simulink model "ASM_AnimationInterface"  (R2024a)
settings: Solver=ode1  StartTime=SIM.tstart.v  StopTime=SIM.tend.v  FixedStep=SIM.StepSize.v  RelTol=1e-3
PostLoadFcn:
  | , if any(exist('dsrtsu_mdlpostloadfcn', 'file') ~= 0), dsrtsu_mdlpostloadfcn('Execute', bdroot); end,
undefined symbols (not defined in the file): a0b2, b98103fe8ad365046cd0, dsmsi, MDL, SIM
libraries: simulink x22, dsmsilib x15, dsmpblib x4, ASM_Environment_lib x1
(part 2 of 7)

== system ASM_AnimationInterface/AnimationInterface/ANIMATION_INTERFACE/ACC_Instruments ==
  DriverAssistance_Animation : Inport
  ACC_Instruments : dsmsilib/dsmsi_simulation_data_objects_BL1  Priority=10001  parameterStr="{\"Version\":1,\"TransformInput\":false,\"EnableInput\":true,\"Objects\":[{\"Name\":\"ACC_State\",\"TypeClass\":{\"Name\":\"Signal\",\"Class\":3,\"SignalProperty\":{\"Description\":null,\"Unit\":null,\"Type\":0,\"Length\":1,\"ObjectsCount\":1},\"TransformationProperty\":null,\"PositionAndScaleProperty\":null,\"PositionProperty\":null},\"Children\":[],\"Oid\":1},{\"Name\":\"ACC_Target_Detected\",\"TypeClass\":{\"Name\":\"Signal\",\"Class\":3,\"SignalProperty\":{\"Description\":null,\"Unit\":null,\"Type\":0,\"Length\":1,\"ObjectsCount\":1},\"TransformationProperty\":null,\"PositionAndScaleProperty\":null,\"PositionProperty\":null},\"Children\":[],\"Oid\":2},{\"Name\":\"ACC_v_Set\",\"TypeClass\":{\"Name\":\"Signal\",\"Class\":3,\"SignalProperty\":{\"Description\":null,\"Unit\":\"km/h\",\"Type\":0,\"Length\":1,\"ObjectsCount\":1},\"TransformationProperty\":null,\"PositionAndScaleProperty\":null,\"PositionProperty\":null},\"Children\":[],\"Oid\":3},{\"Name\":\"ACC_Dist_Set\",\"TypeClass\":{\"Name\":\"Signal\",\"Class\":3,\"SignalProperty\":{\"Description\":null,\"Unit\":\"m\",\"Type\":0,\"Length\":1,\"ObjectsCount\":1},\"TransformationProperty\":null,\"PositionAndScaleProperty\":null,\"PositionProperty\":null},\"Children\":[],\"Oid\":4},{\"Name\":\"ACC_Dist_Target\",\"TypeClass\":{\"Name\":\"Signal\",\"Class\":3,\"SignalProperty\":{\"Description\":null,\"Unit\":\"m\",\"Type\":0,\"Length\":1,\"ObjectsCount\":1},\"TransformationProperty\":null,\"PositionAndScaleProperty\":null,\"PositionProperty\":null},\"Children\":[],\"Oid\":5}]}"  evalStr=dsmsi(gcb, 'EvalJson')  sampleTime=-1  globalBlockId=0  objectsBlockId=dsmsi(gcb, 'GetObjectBlockId')  objectsBlockGuiOpen=dsmsi(gcb, 'GetSdoGuiStatus')  dialogIsOpen=0  blockVersion=60  highPrecision=0  validNameBckp=ACC_Instruments
      settings: SourceProductName=dSPACE MSI Blockset
  Bus Selector7 : BusSelector  OutputSignals=State_ACC[0Off|1On],Target_Detected[0|1],v_Set[km|h],Distance_Set[m],Dist_Long[m]
  Enable_Data_Transfer : Constant
  wires:
  Bus Selector7/3 -> ACC_Instruments/4  "<v_Set[km|h]>"
  Bus Selector7/4 -> ACC_Instruments/5  "<Distance_Set[m]>"
  DriverAssistance_Animation/1 -> Bus Selector7/1
  Bus Selector7/5 -> ACC_Instruments/6  "<Dist_Long[m]>"
  Bus Selector7/1 -> ACC_Instruments/2  "<State_ACC[0Off|1On]>"
  Bus Selector7/2 -> ACC_Instruments/3  "<Target_Detected[0|1]>"
  Enable_Data_Transfer/1 -> ACC_Instruments/1

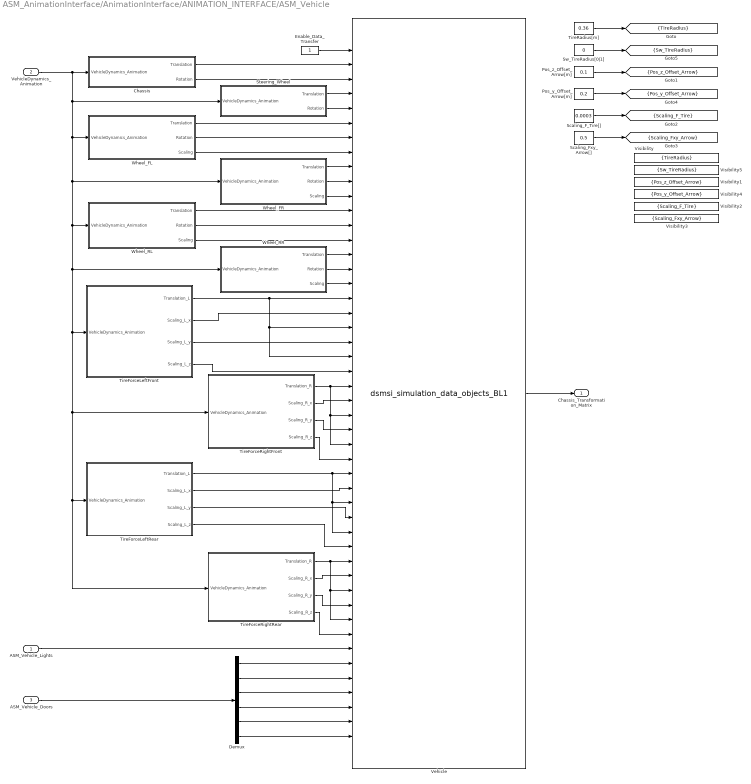
== system ASM_AnimationInterface/AnimationInterface/ANIMATION_INTERFACE/ASM_Vehicle ==
  ASM_Vehicle_Lights : Inport
  VehicleDynamics_Animation : Inport  Port=2
  ASM_Vehicle_Doors : Inport  Port=3
  Chassis : Subsystem
  Demux : Demux  Outputs=6
  Enable_Data_Transfer : Constant
  Pos_y_Offset_Arrow[m] : Constant  Value=0.2
  Pos_z_Offset_Arrow[m] : Constant  Value=0.1
  Scaling_F_Tire[] : Constant  Value=0.0003
  Scaling_Fxy_Arrow[] : Constant  Value=0.5
  Steering_Wheel : Subsystem
  Sw_TireRadius[0|1] : Constant  Value=0
  TireForceLeftFront : Subsystem
  TireForceLeftRear : Subsystem
  TireForceRightFront : Subsystem
  TireForceRightRear : Subsystem
  TireRadius[m] : Constant  Value=0.36
  Vehicle : dsmsilib/dsmsi_simulation_data_objects_BL1  Priority=10001  parameterStr="{\"Version\":1,\"TransformInput\":false,\"EnableInput\":true,\"Objects\":[{\"Oid\":1,\"Name\":\"chassis\",\"TypeClass\":{\"Name\":\"Transformation\",\"Class\":1,\"SignalProperty\":null,\"TransformationProperty\":{\"ObjectsCount\":1,\"TransformMatrixIn\":false,\"TransformMatrixOut\":true,\"AngleInterpretation\":0,\"TransformationOrder\":0,\"RotationOrder\":0,\"TranslationAsParameter\":false,\"Translation\":\"[0 0 0]\",\"RotationAsParameter\":false,\"Rotation\":\"[0 0 0]\",\"ScalingAsParameter\":true,\"Scaling\":\"[1 1 1]\"},\"PositionAndScaleProperty\":null,\"PositionProperty\":null},\"Children\":[{\"Oid\":2,\"Name\":\"steering_wheel\",\"TypeClass\":{\"Name\":\"Transformation\",\"Class\":1,\"SignalProperty\":null,\"TransformationProperty\":{\"ObjectsCount\":1,\"TransformMatrixIn\":false,\"TransformMatrixOut\":false,\"AngleInterpretation\":0,\"TransformationOrder\":0,\"RotationOrder\":0,\"TranslationAsParameter\":false,\"Translation\":\"[0 0 0]\",\"RotationAsParameter\":false,\"Rotation\":\"[0 0 0]\",\"ScalingAsParameter\":true,\"Scaling\":\"[1 1 1]\"},\"PositionAndScaleProperty\":null,\"PositionProperty\":null},\"Children\":[]},{\"Oid\":3,\"Name\":\"wheel_FL\",\"TypeClass\":{\"Name\":\"Transformation\",\"Class\":1,\"SignalProperty\":null,\"TransformationProperty\":{\"ObjectsCount\":1,\"TransformMatrixIn\":false,\"TransformMatrixOut\":false,\"AngleInterpretation\":0,\"TransformationOrder\":0,\"RotationOrder\":1,\"TranslationAsParameter\":false,\"Translation\":\"[0 0 0]\",\"RotationAsParameter\":false,\"Rotation\":\"[0 0 0]\",\"ScalingAsParameter\":false,\"Scaling\":\"[1 1 1]\"},\"PositionAndScaleProperty\":null,\"PositionProperty\":null},\"Children\":[]},{\"Oid\":4,\"Name\":\"wheel_FR\",\"TypeClass\":{\"Name\":\"Transformation\",\"Class\":1,\"SignalProperty\":null,\"TransformationProperty\":{\"ObjectsCount\":1,\"TransformMatrixIn\":false,\"TransformMatrixOut\":false,\"AngleInterpretation\":0,\"TransformationOrder\":0,\"RotationOrder\":1,\"TranslationAsParameter\":false,\"Translation\":\"[0 0 0]\",\"RotationAsParameter\":false,\"Rotation\":\"[0 0 0]\",\"ScalingAsParameter\":false,\"Scaling\":\"[1 1 1]\"},\"PositionAndScaleProperty\":null,\"PositionProperty\":null},\"Children\":[]},{\"Oid\":7,\"Name\":\"wheel_RL\",\"TypeClass\":{\"Name\":\"Transformation\",\"Class\":1,\"SignalProperty\":null,\"TransformationProperty\":{\"ObjectsCount\":1,\"TransformMatrixIn\":false,\"TransformMatrixOut\":false,\"AngleInterpretation\":0,\"TransformationOrder\":0,\"RotationOrder\":1,\"TranslationAsParameter\":false,\"Translation\":\"[0 0 0]\",\"RotationAsParameter\":false,\"Rotation\":\"[0 0 0]\",\"ScalingAsParameter\":false,\"Scaling\":\"[1 1 1]\"},\"PositionAndScaleProperty\":null,\"PositionProperty\":null},\"Children\":[]},{\"Oid\":8,\"Name\":\"wheel_RR\",\"TypeClass\":{\"Name\":\"Transformation\",\"Class\":1,\"SignalProperty\":null,\"TransformationProperty\":{\"ObjectsCount\":1,\"TransformMatrixIn\":false,\"TransformMatrixOut\":false,\"AngleInterpretation\":0,\"TransformationOrder\":0,\"RotationOrder\":1,\"TranslationAsParameter\":false,\"Translation\":\"[0 0 0]\",\"RotationAsParameter\":false,\"Rotation\":\"[0 0 0]\",\"ScalingAsParameter\":false,\"Scaling\":\"[1 1 1]\"},\"PositionAndScaleProperty\":null,\"PositionProperty\":null},\"Children\":[]},{\"Oid\":5,\"Name\":\"_TireFrcs_F_L_x\",\"TypeClass\":{\"Name\":\"Transformation\",\"Class\":1,\"SignalProperty\":null,\"TransformationProperty\":{\"ObjectsCount\":1,\"TransformMatrixIn\":false,\"TransformMatrixOut\":false,\"AngleInterpretation\":0,\"TransformationOrder\":0,\"RotationOrder\":0,\"TranslationAsParameter\":false,\"Translation\":\"[0 0 0]\",\"RotationAsParameter\":true,\"Rotation\":\"[0 90 0]\",\"ScalingAsParameter\":false,\"Scaling\":\"[1 1 1]\"},\"PositionAndScaleProperty\":null,\"PositionProperty\":null},\"Children\":[]},{\"Oid\":12,\"Name\":\"_TireFrcs_F_L_y\",\"TypeClass\":{\"Name\":\"Transformation\",\"Class\":1,\"SignalProperty\":null,\"TransformationProperty\":{\"ObjectsCount\":1,\"TransformMatrixIn\":false,\"TransformMatrixOut\":false,\"AngleInterpretation\":0,\"TransformationOrder\":0,\"RotationOrder\":0,\"TranslationAsParameter\":false,\"Translation\":\"[0 0 0]\",\"RotationAsParameter\":true,\"Rotation\":\"[0 0 -90]\",\"ScalingAsParameter\":false,\"Scaling\":\"[1 1 1]\"},\"PositionAndScaleProperty\":null,\"PositionProperty\":null},\"Children\":[]},{\"Oid\":13,\"Name\":\"_TireFrcs_F_L_z\",\"TypeClass\":{\"Name\":\"Transformation\",\"Class\":1,\"SignalProperty\":null,\"TransformationProperty\":{\"ObjectsCount\":1,\"TransformMatrixIn\":false,\"TransformMatrixOut\":false,\"AngleInterpretation\":0,\"TransformationOrder\":0,\"RotationOrder\":0,\"TranslationAsParameter\":false,\"Translation\":\"[0 0 0]\",\"RotationAsParameter\":true,\"Rotation\":\"[0 0 0]\",\"ScalingAsParameter\":false,\"Scaling\":\"[1 1 1]\"},\"PositionAndScaleProperty\":null,\"PositionProperty\":null},\"Children\":[]},{\"Oid\":6,\"Name\":\"_TireFrcs_F_R_x\",\"TypeClass\":{\"Name\":\"Transformation\",\"Class\":1,\"SignalProperty\":null,\"TransformationProperty\":{\"ObjectsCount\":1,\"TransformMatrixIn\":false,\"TransformMatrixOut\":false,\"AngleInterpretation\":0,\"TransformationOrder\":0,\"RotationOrder\":0,\"TranslationAsParameter\":false,\"Translation\":\"[0 0 0]\",\"RotationAsParameter\":true,\"Rotation\":\"[0 90 0]\",\"ScalingAsParameter\":false,\"Scaling\":\"[1 1 1]\"},\"PositionAndScaleProperty\":null,\"PositionProperty\":null},\"Children\":[]},{\"Oid\":14,\"Name\":\"_TireFrcs_F_R_y\",\"TypeClass\":{\"Name\":\"Transformation\",\"Class\":1,\"SignalProperty\":null,\"TransformationProperty\":{\"ObjectsCount\":1,\"TransformMatrixIn\":false,\"TransformMatrixOut\":false,\"AngleInterpretation\":0,\"TransformationOrder\":0,\"RotationOrder\":0,\"TranslationAsParameter\":false,\"Translation\":\"[0 0 0]\",\"RotationAsParameter\":true,\"Rotation\":\"[0 0 -90]\",\"ScalingAsParameter\":false,\"Scaling\":\"[1 1 1]\"},\"PositionAndScaleProperty\":null,\"PositionProperty\":null},\"Children\":[]},{\"Oid\":15,\"Name\":\"_TireFrcs_F_R_z\",\"TypeClass\":{\"Name\":\"Transformation\",\"Class\":1,\"SignalProperty\":null,\"TransformationProperty\":{\"ObjectsCount\":1,\"TransformMatrixIn\":false,\"TransformMatrixOut\":false,\"AngleInterpretation\":0,\"TransformationOrder\":0,\"RotationOrder\":0,\"TranslationAsParameter\":false,\"Translation\":\"[0 0 0]\",\"RotationAsParameter\":true,\"Rotation\":\"[0 0 0]\",\"ScalingAsParameter\":false,\"Scaling\":\"[1 1 1]\"},\"PositionAndScaleProperty\":null,\"PositionProperty\":null},\"Children\":[]},{\"Oid\":9,\"Name\":\"_TireFrcs_R_L_x\",\"TypeClass\":{\"Name\":\"Transformation\",\"Class\":1,\"SignalProperty\":null,\"TransformationProperty\":{\"ObjectsCount\":1,\"TransformMatrixIn\":false,\"TransformMatrixOut\":false,\"AngleInterpretation\":0,\"TransformationOrder\":0,\"RotationOrder\":0,\"TranslationAsParameter\":false,\"Translation\":\"[0 0 0]\",\"RotationAsParameter\":true,\"Rotation\":\"[0 90 0]\",\"ScalingAsParameter\":false,\"Scaling\":\"[1 1 1]\"},\"PositionAndScaleProperty\":null,\"PositionProperty\":null},\"Children\":[]},{\"Oid\":16,\"Name\":\"_TireFrcs_R_L_y\",\"TypeClass\":{\"Name\":\"Transformation\",\"Class\":1,\"SignalProperty\":null,\"TransformationProperty\":{\"ObjectsCount\":1,\"TransformMatrixIn\":false,\"TransformMatrixOut\":false,\"AngleInterpretation\":0,\"TransformationOrder\":0,\"RotationOrder\":0,\"TranslationAsParameter\":false,\"Translation\":\"[0 0 0]\",\"RotationAsParameter\":true,\"Rotation\":\"[0 0 -90]\",\"ScalingAsParameter\":false,\"Scaling\":\"[1 1 1]\"},\"PositionAndScaleProperty\":null,\"PositionProperty\":null},\"Children\":[]},{\"Oid\":17,\"Name\":\"_TireFrcs_R_L_z\",\"TypeClass\":{\"Name\":\"Transformation\",\"Class\":1,\"SignalProperty\":null,\"TransformationProperty\":{\"ObjectsCount\":1,\"TransformMatrixIn\":false,\"TransformMatrixOut\":false,\"AngleInterpretation\":0,\"TransformationOrder\":0,\"RotationOrder\":0,\"TranslationAsParameter\":false,\"Translation\":\"[0 0 0]\",\"RotationAsParameter\":true,\"Rotation\":\"[0 0 0]\",\"ScalingAsParameter\":false,\"Scaling\":\"[1 1 1]\"},\"PositionAndScaleProperty\":null,\"PositionProperty\":null},\"Children\":[]},{\"Oid\":10,\"Name\":\"_TireFrcs_R_R_x\",\"TypeClass\":{\"Name\":\"Transformation\",\"Class\":1,\"SignalProperty\":null,\"TransformationProperty\":{\"ObjectsCount\":1,\"TransformMatrixIn\":false,\"TransformMatrixOut\":false,\"AngleInterpretation\":0,\"TransformationOrder\":0,\"RotationOrder\":0,\"TranslationAsParameter\":false,\"Translation\":\"[0 0 0]\",\"RotationAsParameter\":true,\"Rotation\":\"[0 90 0]\",\"ScalingAsParameter\":false,\"Scaling\":\"[1 1 1]\"},\"PositionAndScaleProperty\":null,\"PositionProperty\":null},\"Children\":[]},{\"Oid\":18,\"Name\":\"_TireFrcs_R_R_y\",\"TypeClass\":{\"Name\":\"Transformation\",\"Class\":1,\"SignalProperty\":null,\"TransformationProperty\":{\"ObjectsCount\":1,\"TransformMatrixIn\":false,\"TransformMatrixOut\":false,\"AngleInterpretation\":0,\"TransformationOrder\":0,\"RotationOrder\":0,\"TranslationAsParameter\":false,\"Translation\":\"[0 0 0]\",\"RotationAsParameter\":true,\"Rotation\":\"[0 0 -90]\",\"ScalingAsParameter\":false,\"Scaling\":\"[1 1 1]\"},\"PositionAndScaleProperty\":null,\"PositionProperty\":null},\"Children\":[]},{\"Oid\":19,\"Name\":\"_TireFrcs_R_R_z\",\"TypeClass\":{\"Name\":\"Transformation\",\"Class\":1,\"SignalProperty\":null,\"TransformationProperty\":{\"ObjectsCount\":1,\"TransformMatrixIn\":false,\"TransformMatrixOut\":false,\"AngleInterpretation\":0,\"TransformationOrder\":0,\"RotationOrder\":0,\"TranslationAsParameter\":false,\"Translation\":\"[0 0 0]\",\"RotationAsParameter\":true,\"Rotation\":\"[0 0 0]\",\"ScalingAsParameter\":false,\"Scaling\":\"[1 1 1]\"},\"PositionAndScaleProperty\":null,\"PositionProperty\":null},\"Children\":[]},{\"Oid\":11,\"Name\":\"ASM_Vehicle_Lights\",\"TypeClass\":{\"Name\":\"Signal\",\"Class\":3,\"SignalProperty\":{\"ObjectsCount\":1,\"InstrumentInput\":\"Input port\",\"Description\":null,\"Unit\":null,\"Type\":7,\"Length\":1},\"TransformationProperty\":null,\"PositionAndScaleProperty\":null,\"PositionProperty\":null},\"Children\":[]},{\"Oid\":21,\"Name\":\"Door_FL\",\"TypeClass\":{\"Name\":\"Signal\",\"Class\":3,\"SignalProperty\":{\"ObjectsCount\":1,\"InstrumentInput\":\"Input port\",\"Description\":null,\"Unit\":null,\"Type\":0,\"Length\":1},\"TransformationProperty\":null,\"PositionAndScaleProperty\":null,\"PositionProperty\":null},\"Children\":[]},{\"Oid\":22,\"Name\":\"Door_FR\",\"TypeClass\":{\"Name\":\"Signal\",\"Class\":3,\"SignalProperty\":{\"ObjectsCount\":1,\"InstrumentInput\":\"Input port\",\"Description\":null,\"Unit\":null,\"Type\":0,\"Length\":1},\"TransformationProperty\":null,\"PositionAndScaleProperty\":null,\"PositionProperty\":null},\"Children\":[]},{\"Oid\":23,\"Name\":\"Door_RL\",\"TypeClass\":{\"Name\":\"Signal\",\"Class\":3,\"SignalProperty\":{\"ObjectsCount\":1,\"InstrumentInput\":\"Input port\",\"Description\":null,\"Unit\":null,\"Type\":0,\"Length\":1},\"TransformationProperty\":null,\"PositionAndScaleProperty\":null,\"PositionProperty\":null},\"Children\":[]},{\"Oid\":24,\"Name\":\"Door_RR\",\"TypeClass\":{\"Name\":\"Signal\",\"Class\":3,\"SignalProperty\":{\"ObjectsCount\":1,\"InstrumentInput\":\"Input port\",\"Description\":null,\"Unit\":null,\"Type\":0,\"Length\":1},\"TransformationProperty\":null,\"PositionAndScaleProperty\":null,\"PositionProperty\":null},\"Children\":[]},{\"Oid\":25,\"Name\":\"Hood\",\"TypeClass\":{\"Name\":\"Signal\",\"Class\":3,\"SignalProperty\":{\"ObjectsCount\":1,\"InstrumentInput\":\"Input port\",\"Description\":null,\"Unit\":null,\"Type\":0,\"Length\":1},\"TransformationProperty\":null,\"PositionAndScaleProperty\":null,\"PositionProperty\":null},\"Children\":[]},{\"Oid\":26,\"Name\":\"Trunk\",\"TypeClass\":{\"Name\":\"Signal\",\"Class\":3,\"SignalProperty\":{\"ObjectsCount\":1,\"InstrumentInput\":\"Input port\",\"Description\":null,\"Unit\":null,\"Type\":0,\"Length\":1},\"TransformationProperty\":null,\"PositionAndScaleProperty\":null,\"PositionProperty\":null},\"Children\":[]}]}]}"  evalStr=dsmsi(gcb, 'EvalJson')  sampleTime=-1  globalBlockId=0  objectsBlockId=dsmsi(gcb, 'GetObjectBlockId')  objectsBlockGuiOpen=dsmsi(gcb, 'GetSdoGuiStatus')  dialogIsOpen=0  blockVersion=60  highPrecision=0  validNameBckp=Vehicle
      settings: SourceProductName=dSPACE MSI Blockset
  Visibility : GotoTagVisibility  GotoTag=TireRadius
  Visibility1 : GotoTagVisibility  GotoTag=Pos_z_Offset_Arrow
  Visibility2 : GotoTagVisibility  GotoTag=Scaling_F_Tire
  Visibility3 : GotoTagVisibility  GotoTag=Scaling_Fxy_Arrow
  Visibility4 : GotoTagVisibility  GotoTag=Pos_y_Offset_Arrow
  Visibility5 : GotoTagVisibility  GotoTag=Sw_TireRadius
  Wheel_FL : Subsystem
  Wheel_FR : Subsystem
  Wheel_RL : Subsystem
  Wheel_RR : Subsystem
  Chassis_Transformation_Matrix : Outport
  tag scope: Pos_y_Offset_Arrow=scoped, Pos_z_Offset_Arrow=scoped, Scaling_F_Tire=scoped, Scaling_Fxy_Arrow=scoped, Sw_TireRadius=scoped, TireRadius=scoped
  wires:
  Vehicle/1 -> Chassis_Transformation_Matrix/1
  VehicleDynamics_Animation/1 -> Wheel_FL/1(VehicleDynamics_Animation), Wheel_FR/1(VehicleDynamics_Animation), Wheel_RR/1(VehicleDynamics_Animation), TireForceRightRear/1(VehicleDynamics_Animation), TireForceLeftRear/1(VehicleDynamics_Animation), TireForceRightFront/1(VehicleDynamics_Animation), TireForceLeftFront/1(VehicleDynamics_Animation), Wheel_RL/1(VehicleDynamics_Animation), Steering_Wheel/1(VehicleDynamics_Animation), Chassis/1(VehicleDynamics_Animation)
  ASM_Vehicle_Doors/1 -> Demux/1
  Scaling_F_Tire[]/1 -> [Scaling_F_Tire]
  Sw_TireRadius[0|1]/1 -> [Sw_TireRadius]
  Pos_z_Offset_Arrow[m]/1 -> [Pos_z_Offset_Arrow]
  Scaling_Fxy_Arrow[]/1 -> [Scaling_Fxy_Arrow]
  Pos_y_Offset_Arrow[m]/1 -> [Pos_y_Offset_Arrow]
  TireRadius[m]/1 -> [TireRadius]
  TireForceRightRear/4(Scaling_R_z) -> Vehicle/41
  TireForceRightRear/3(Scaling_R_y) -> Vehicle/39
  TireForceRightRear/2(Scaling_R_x) -> Vehicle/37
  TireForceRightRear/1(Translation_R) -> Vehicle/38, Vehicle/40, Vehicle/36
  TireForceLeftRear/4(Scaling_L_z) -> Vehicle/35
  TireForceLeftRear/3(Scaling_L_y) -> Vehicle/33
  TireForceLeftRear/2(Scaling_L_x) -> Vehicle/31
  TireForceLeftRear/1(Translation_L) -> Vehicle/34, Vehicle/32, Vehicle/30
  ASM_Vehicle_Lights/1 -> Vehicle/42
  Chassis/1(Translation) -> Vehicle/2
  Chassis/2(Rotation) -> Vehicle/3
  Steering_Wheel/1(Translation) -> Vehicle/4
  Steering_Wheel/2(Rotation) -> Vehicle/5
  Wheel_FL/2(Rotation) -> Vehicle/7
  Wheel_FL/3(Scaling) -> Vehicle/8
  Wheel_FL/1(Translation) -> Vehicle/6
  Wheel_FR/1(Translation) -> Vehicle/9
  Wheel_FR/2(Rotation) -> Vehicle/10
  Wheel_FR/3(Scaling) -> Vehicle/11
  Wheel_RL/1(Translation) -> Vehicle/12
  Wheel_RL/2(Rotation) -> Vehicle/13
  Wheel_RL/3(Scaling) -> Vehicle/14
  Wheel_RR/1(Translation) -> Vehicle/15
  Wheel_RR/2(Rotation) -> Vehicle/16
  Wheel_RR/3(Scaling) -> Vehicle/17
  Enable_Data_Transfer/1 -> Vehicle/1
  TireForceLeftFront/1(Translation_L) -> Vehicle/22, Vehicle/20, Vehicle/18
  TireForceLeftFront/2(Scaling_L_x) -> Vehicle/19
  TireForceLeftFront/3(Scaling_L_y) -> Vehicle/21
  TireForceLeftFront/4(Scaling_L_z) -> Vehicle/23
  TireForceRightFront/1(Translation_R) -> Vehicle/28, Vehicle/26, Vehicle/24
  TireForceRightFront/2(Scaling_R_x) -> Vehicle/25
  TireForceRightFront/3(Scaling_R_y) -> Vehicle/27
  TireForceRightFront/4(Scaling_R_z) -> Vehicle/29
  Demux/1 -> Vehicle/43
  Demux/2 -> Vehicle/44
  Demux/3 -> Vehicle/45
  Demux/4 -> Vehicle/46
  Demux/5 -> Vehicle/47
  Demux/6 -> Vehicle/48

== system ASM_AnimationInterface/AnimationInterface/ANIMATION_INTERFACE/ASM_Vehicle_Instruments ==
  VehicleDynamics_Animation : Inport
  Environment_Animation : Inport  Port=2
  Drivetrain_Animation : Inport  Port=3
  Bus Selector1 : BusSelector  OutputSignals=v_x_Vehicle_CoG[km|h],a_y_Vehicle_CoG[m|s2],YawRate_Vehicle_CoG[deg|s]
  Bus Selector15 : BusSelector  OutputSignals=n_Engine[rpm],Gear[]
  Bus Selector2 : BusSelector  OutputSignals=s_Vehicle[m],Angle_Yaw_Vehicle_CoorSys_E[deg]
  Bus Selector4 : BusSelector  OutputSignals=s_Veh_Road[m],ManeuverTime[s],ManeuverState[]
  Enable_Data_Transfer : Constant
  Vehicle_Instruments : dsmsilib/dsmsi_simulation_data_objects_BL1  Priority=10001  parameterStr="{\"Version\":1,\"TransformInput\":false,\"EnableInput\":true,\"Objects\":[{\"Oid\":1,\"Name\":\"Speed\",\"TypeClass\":{\"Name\":\"Signal\",\"Class\":3,\"SignalProperty\":{\"InstrumentInput\":\"Input port\",\"Description\":null,\"Unit\":\"km/h\",\"Type\":0,\"Length\":1,\"ObjectsCount\":1},\"TransformationProperty\":null,\"PositionAndScaleProperty\":null,\"PositionProperty\":null},\"Children\":[]},{\"Oid\":2,\"Name\":\"LatAcc\",\"TypeClass\":{\"Name\":\"Signal\",\"Class\":3,\"SignalProperty\":{\"InstrumentInput\":\"Input port\",\"Description\":null,\"Unit\":\"m/s2\",\"Type\":0,\"Length\":1,\"ObjectsCount\":1},\"TransformationProperty\":null,\"PositionAndScaleProperty\":null,\"PositionProperty\":null},\"Children\":[]},{\"Oid\":3,\"Name\":\"YawRate\",\"TypeClass\":{\"Name\":\"Signal\",\"Class\":3,\"SignalProperty\":{\"InstrumentInput\":\"Input port\",\"Description\":null,\"Unit\":\"deg/s\",\"Type\":0,\"Length\":1,\"ObjectsCount\":1},\"TransformationProperty\":null,\"PositionAndScaleProperty\":null,\"PositionProperty\":null},\"Children\":[]},{\"Oid\":4,\"Name\":\"Engine\",\"TypeClass\":{\"Name\":\"Signal\",\"Class\":3,\"SignalProperty\":{\"InstrumentInput\":\"Input port\",\"Description\":null,\"Unit\":\"rpm\",\"Type\":0,\"Length\":1,\"ObjectsCount\":1},\"TransformationProperty\":null,\"PositionAndScaleProperty\":null,\"PositionProperty\":null},\"Children\":[]},{\"Oid\":5,\"Name\":\"Gear\",\"TypeClass\":{\"Name\":\"Signal\",\"Class\":3,\"SignalProperty\":{\"InstrumentInput\":\"Input port\",\"Description\":null,\"Unit\":null,\"Type\":0,\"Length\":1,\"ObjectsCount\":1},\"TransformationProperty\":null,\"PositionAndScaleProperty\":null,\"PositionProperty\":null},\"Children\":[]},{\"Oid\":6,\"Name\":\"s_Road\",\"TypeClass\":{\"Name\":\"Signal\",\"Class\":3,\"SignalProperty\":{\"InstrumentInput\":\"Input port\",\"Description\":null,\"Unit\":\"m\",\"Type\":0,\"Length\":1,\"ObjectsCount\":1},\"TransformationProperty\":null,\"PositionAndScaleProperty\":null,\"PositionProperty\":null},\"Children\":[]},{\"Oid\":7,\"Name\":\"ManeuverTime\",\"TypeClass\":{\"Name\":\"Signal\",\"Class\":3,\"SignalProperty\":{\"InstrumentInput\":\"Input port\",\"Description\":null,\"Unit\":\"s\",\"Type\":0,\"Length\":1,\"ObjectsCount\":1},\"TransformationProperty\":null,\"PositionAndScaleProperty\":null,\"PositionProperty\":null},\"Children\":[]},{\"Oid\":8,\"Name\":\"ManeuverState\",\"TypeClass\":{\"Name\":\"Signal\",\"Class\":3,\"SignalProperty\":{\"InstrumentInput\":\"Input port\",\"Description\":null,\"Unit\":null,\"Type\":0,\"Length\":1,\"ObjectsCount\":1},\"TransformationProperty\":null,\"PositionAndScaleProperty\":null,\"PositionProperty\":null},\"Children\":[]},{\"Oid\":9,\"Name\":\"DrivenDistance\",\"TypeClass\":{\"Name\":\"Signal\",\"Class\":3,\"SignalProperty\":{\"InstrumentInput\":\"Input port\",\"Description\":null,\"Unit\":\"m\",\"Type\":0,\"Length\":1,\"ObjectsCount\":1},\"TransformationProperty\":null,\"PositionAndScaleProperty\":null,\"PositionProperty\":null},\"Children\":[]},{\"Oid\":10,\"Name\":\"YawAngle\",\"TypeClass\":{\"Name\":\"Signal\",\"Class\":3,\"SignalProperty\":{\"InstrumentInput\":\"Input port\",\"Description\":null,\"Unit\":\"deg\",\"Type\":0,\"Length\":1,\"ObjectsCount\":1},\"TransformationProperty\":null,\"PositionAndScaleProperty\":null,\"PositionProperty\":null},\"Children\":[]}]}"  evalStr=dsmsi(gcb, 'EvalJson')  sampleTime=-1  globalBlockId=0  objectsBlockId=dsmsi(gcb, 'GetObjectBlockId')  objectsBlockGuiOpen=dsmsi(gcb, 'GetSdoGuiStatus')  dialogIsOpen=0  blockVersion=60  highPrecision=0  validNameBckp=Vehicle_Instruments
      settings: SourceProductName=dSPACE MSI Blockset
  wires:
  Bus Selector15/2 -> Vehicle_Instruments/6  "<Gear[]>"
  Bus Selector15/1 -> Vehicle_Instruments/5  "<n_Engine[rpm]>"
  Drivetrain_Animation/1 -> Bus Selector15/1
  VehicleDynamics_Animation/1 -> Bus Selector2/1, Bus Selector1/1
  Bus Selector4/3 -> Vehicle_Instruments/9  "<ManeuverState[]>"
  Bus Selector1/3 -> Vehicle_Instruments/4  "<YawRate_Vehicle_CoG[deg|s]>"
  Bus Selector1/1 -> Vehicle_Instruments/2  "<v_x_Vehicle_CoG[km|h]>"
  Bus Selector1/2 -> Vehicle_Instruments/3  "<a_y_Vehicle_CoG[m|s2]>"
  Bus Selector4/2 -> Vehicle_Instruments/8  "<ManeuverTime[s]>"
  Bus Selector4/1 -> Vehicle_Instruments/7  "<s_Veh_Road[m]>"
  Bus Selector2/1 -> Vehicle_Instruments/10  "<s_Vehicle[m]>"
  Bus Selector2/2 -> Vehicle_Instruments/11  "<Angle_Yaw_Vehicle_CoorSys_E[deg]>"
  Environment_Animation/1 -> Bus Selector4/1
  Enable_Data_Transfer/1 -> Vehicle_Instruments/1

== system ASM_AnimationInterface/AnimationInterface/ANIMATION_INTERFACE/ASM_Vehicle_Occupants ==
  Environment_Animation : Inport
  Bus Selector : BusSelector  OutputSignals=UserSignals_Customized.DriverMonitoring.DriverGazeLocation[],UserSignals_Customized.DriverMonitoring.DriverAnimation[],UserSignals_Customized.DriverMonitoring.DriverLizardOwlRatio[]
  Enable_Data_Transfer : Constant
  Vehicle_Occupants : dsmsilib/dsmsi_simulation_data_objects_BL1  Priority=10001  parameterStr="{\"Version\":1,\"TransformInput\":false,\"EnableInput\":true,\"Objects\":[{\"Oid\":1,\"Name\":\"Driver\",\"TypeClass\":{\"Name\":\"Transformation\",\"Class\":1,\"SignalProperty\":null,\"TransformationProperty\":{\"ObjectsCount\":1,\"TransformMatrixIn\":false,\"TransformMatrixOut\":false,\"AngleInterpretation\":0,\"TransformationOrder\":0,\"RotationOrder\":0,\"TranslationAsParameter\":true,\"Translation\":\"[0 0 0]\",\"RotationAsParameter\":true,\"Rotation\":\"[0 0 0]\",\"ScalingAsParameter\":true,\"Scaling\":\"[1 1 1]\"},\"PositionAndScaleProperty\":null,\"PositionProperty\":null},\"Children\":[{\"Oid\":2,\"Name\":\"DMS_GazeLocation\",\"TypeClass\":{\"Name\":\"Signal\",\"Class\":3,\"SignalProperty\":{\"ObjectsCount\":1,\"InstrumentInput\":\"Input port\",\"Description\":null,\"Unit\":null,\"Type\":0,\"Length\":1},\"TransformationProperty\":null,\"PositionAndScaleProperty\":null,\"PositionProperty\":null},\"Children\":[]},{\"Oid\":3,\"Name\":\"DMS_DriverAnimation\",\"TypeClass\":{\"Name\":\"Signal\",\"Class\":3,\"SignalProperty\":{\"ObjectsCount\":1,\"InstrumentInput\":\"Input port\",\"Description\":null,\"Unit\":null,\"Type\":0,\"Length\":1},\"TransformationProperty\":null,\"PositionAndScaleProperty\":null,\"PositionProperty\":null},\"Children\":[]},{\"Oid\":4,\"Name\":\"DMS_LizardOwlRatio\",\"TypeClass\":{\"Name\":\"Signal\",\"Class\":3,\"SignalProperty\":{\"ObjectsCount\":1,\"InstrumentInput\":\"Input port\",\"Description\":null,\"Unit\":null,\"Type\":0,\"Length\":1},\"TransformationProperty\":null,\"PositionAndScaleProperty\":null,\"PositionProperty\":null},\"Children\":[]}]}]}"  evalStr=dsmsi(gcb, 'EvalJson')  sampleTime=-1  globalBlockId=0  objectsBlockId=dsmsi(gcb, 'GetObjectBlockId')  objectsBlockGuiOpen=dsmsi(gcb, 'GetSdoGuiStatus')  dialogIsOpen=0  blockVersion=60  highPrecision=0  validNameBckp=Vehicle_Occupants
      settings: SourceProductName=dSPACE MSI Blockset
  wires:
  Environment_Animation/1 -> Bus Selector/1
  Enable_Data_Transfer/1 -> Vehicle_Occupants/1
  Bus Selector/1 -> Vehicle_Occupants/2  "<DriverGazeLocation[]>"
  Bus Selector/2 -> Vehicle_Occupants/3  "<DriverAnimation[]>"
  Bus Selector/3 -> Vehicle_Occupants/4  "<DriverLizardOwlRatio[]>"

== system ASM_AnimationInterface/AnimationInterface/ANIMATION_INTERFACE/Activate_Animation ==

== system ASM_AnimationInterface/AnimationInterface/ANIMATION_INTERFACE/Activate_Animation1 ==

== system ASM_AnimationInterface/AnimationInterface/ANIMATION_INTERFACE/Activate_Animation2 ==

== system ASM_AnimationInterface/AnimationInterface/ANIMATION_INTERFACE/Activate_Animation3 ==

== system ASM_AnimationInterface/AnimationInterface/ANIMATION_INTERFACE/Activate_Animation4 ==

== system ASM_AnimationInterface/AnimationInterface/ANIMATION_INTERFACE/Activate_Animation5 ==

== system ASM_AnimationInterface/AnimationInterface/ANIMATION_INTERFACE/Activate_Animation6 ==

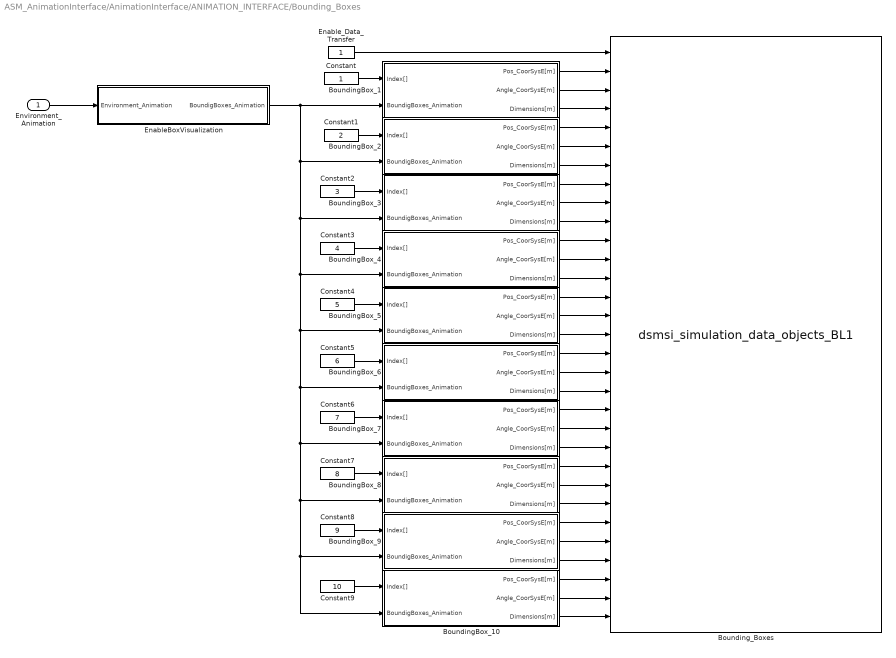
== system ASM_AnimationInterface/AnimationInterface/ANIMATION_INTERFACE/Bounding_Boxes ==
  Environment_Animation : Inport
  BoundingBox_1 : Subsystem
  BoundingBox_10 : Subsystem
  BoundingBox_2 : Subsystem
  BoundingBox_3 : Subsystem
  BoundingBox_4 : Subsystem
  BoundingBox_5 : Subsystem
  BoundingBox_6 : Subsystem
  BoundingBox_7 : Subsystem
  BoundingBox_8 : Subsystem
  BoundingBox_9 : Subsystem
  Bounding_Boxes : dsmsilib/dsmsi_simulation_data_objects_BL1  Priority=10001  parameterStr="{\"Version\":1,\"TransformInput\":false,\"EnableInput\":true,\"Objects\":[{\"Name\":\"Boundingbox_01\",\"TypeClass\":{\"Name\":\"Transformation\",\"Class\":1,\"SignalProperty\":null,\"TransformationProperty\":{\"TransformMatrixIn\":false,\"TransformMatrixOut\":false,\"AngleInterpretation\":0,\"TransformationOrder\":0,\"RotationOrder\":0,\"TranslationAsParameter\":false,\"Translation\":\"[0 0 0]\",\"RotationAsParameter\":false,\"Rotation\":\"[0 0 0]\",\"ScalingAsParameter\":false,\"Scaling\":\"[1 1 1]\",\"ObjectsCount\":1},\"PositionAndScaleProperty\":null,\"PositionProperty\":null},\"Children\":[],\"Oid\":1},{\"Name\":\"Boundingbox_02\",\"TypeClass\":{\"Name\":\"Transformation\",\"Class\":1,\"SignalProperty\":null,\"TransformationProperty\":{\"TransformMatrixIn\":false,\"TransformMatrixOut\":false,\"AngleInterpretation\":0,\"TransformationOrder\":0,\"RotationOrder\":0,\"TranslationAsParameter\":false,\"Translation\":\"[0 0 0]\",\"RotationAsParameter\":false,\"Rotation\":\"[0 0 0]\",\"ScalingAsParameter\":false,\"Scaling\":\"[1 1 1]\",\"ObjectsCount\":1},\"PositionAndScaleProperty\":null,\"PositionProperty\":null},\"Children\":[],\"Oid\":2},{\"Name\":\"Boundingbox_03\",\"TypeClass\":{\"Name\":\"Transformation\",\"Class\":1,\"SignalProperty\":null,\"TransformationProperty\":{\"TransformMatrixIn\":false,\"TransformMatrixOut\":false,\"AngleInterpretation\":0,\"TransformationOrder\":0,\"RotationOrder\":0,\"TranslationAsParameter\":false,\"Translation\":\"[0 0 0]\",\"RotationAsParameter\":false,\"Rotation\":\"[0 0 0]\",\"ScalingAsParameter\":false,\"Scaling\":\"[1 1 1]\",\"ObjectsCount\":1},\"PositionAndScaleProperty\":null,\"PositionProperty\":null},\"Children\":[],\"Oid\":3},{\"Name\":\"Boundingbox_04\",\"TypeClass\":{\"Name\":\"Transformation\",\"Class\":1,\"SignalProperty\":null,\"TransformationProperty\":{\"TransformMatrixIn\":false,\"TransformMatrixOut\":false,\"AngleInterpretation\":0,\"TransformationOrder\":0,\"RotationOrder\":0,\"TranslationAsParameter\":false,\"Translation\":\"[0 0 0]\",\"RotationAsParameter\":false,\"Rotation\":\"[0 0 0]\",\"ScalingAsParameter\":false,\"Scaling\":\"[1 1 1]\",\"ObjectsCount\":1},\"PositionAndScaleProperty\":null,\"PositionProperty\":null},\"Children\":[],\"Oid\":4},{\"Name\":\"Boundingbox_05\",\"TypeClass\":{\"Name\":\"Transformation\",\"Class\":1,\"SignalProperty\":null,\"TransformationProperty\":{\"TransformMatrixIn\":false,\"TransformMatrixOut\":false,\"AngleInterpretation\":0,\"TransformationOrder\":0,\"RotationOrder\":0,\"TranslationAsParameter\":false,\"Translation\":\"[0 0 0]\",\"RotationAsParameter\":false,\"Rotation\":\"[0 0 0]\",\"ScalingAsParameter\":false,\"Scaling\":\"[1 1 1]\",\"ObjectsCount\":1},\"PositionAndScaleProperty\":null,\"PositionProperty\":null},\"Children\":[],\"Oid\":5},{\"Name\":\"Boundingbox_06\",\"TypeClass\":{\"Name\":\"Transformation\",\"Class\":1,\"SignalProperty\":null,\"TransformationProperty\":{\"TransformMatrixIn\":false,\"TransformMatrixOut\":false,\"AngleInterpretation\":0,\"TransformationOrder\":0,\"RotationOrder\":0,\"TranslationAsParameter\":false,\"Translation\":\"[0 0 0]\",\"RotationAsParameter\":false,\"Rotation\":\"[0 0 0]\",\"ScalingAsParameter\":false,\"Scaling\":\"[1 1 1]\",\"ObjectsCount\":1},\"PositionAndScaleProperty\":null,\"PositionProperty\":null},\"Children\":[],\"Oid\":6},{\"Name\":\"Boundingbox_07\",\"TypeClass\":{\"Name\":\"Transformation\",\"Class\":1,\"SignalProperty\":null,\"TransformationProperty\":{\"TransformMatrixIn\":false,\"TransformMatrixOut\":false,\"AngleInterpretation\":0,\"TransformationOrder\":0,\"RotationOrder\":0,\"TranslationAsParameter\":false,\"Translation\":\"[0 0 0]\",\"RotationAsParameter\":false,\"Rotation\":\"[0 0 0]\",\"ScalingAsParameter\":false,\"Scaling\":\"[1 1 1]\",\"ObjectsCount\":1},\"PositionAndScaleProperty\":null,\"PositionProperty\":null},\"Children\":[],\"Oid\":7},{\"Name\":\"Boundingbox_08\",\"TypeClass\":{\"Name\":\"Transformation\",\"Class\":1,\"SignalProperty\":null,\"TransformationProperty\":{\"TransformMatrixIn\":false,\"TransformMatrixOut\":false,\"AngleInterpretation\":0,\"TransformationOrder\":0,\"RotationOrder\":0,\"TranslationAsParameter\":false,\"Translation\":\"[0 0 0]\",\"RotationAsParameter\":false,\"Rotation\":\"[0 0 0]\",\"ScalingAsParameter\":false,\"Scaling\":\"[1 1 1]\",\"ObjectsCount\":1},\"PositionAndScaleProperty\":null,\"PositionProperty\":null},\"Children\":[],\"Oid\":8},{\"Name\":\"Boundingbox_09\",\"TypeClass\":{\"Name\":\"Transformation\",\"Class\":1,\"SignalProperty\":null,\"TransformationProperty\":{\"TransformMatrixIn\":false,\"TransformMatrixOut\":false,\"AngleInterpretation\":0,\"TransformationOrder\":0,\"RotationOrder\":0,\"TranslationAsParameter\":false,\"Translation\":\"[0 0 0]\",\"RotationAsParameter\":false,\"Rotation\":\"[0 0 0]\",\"ScalingAsParameter\":false,\"Scaling\":\"[1 1 1]\",\"ObjectsCount\":1},\"PositionAndScaleProperty\":null,\"PositionProperty\":null},\"Children\":[],\"Oid\":9},{\"Name\":\"Boundingbox_10\",\"TypeClass\":{\"Name\":\"Transformation\",\"Class\":1,\"SignalProperty\":null,\"TransformationProperty\":{\"TransformMatrixIn\":false,\"TransformMatrixOut\":false,\"AngleInterpretation\":0,\"TransformationOrder\":0,\"RotationOrder\":0,\"TranslationAsParameter\":false,\"Translation\":\"[0 0 0]\",\"RotationAsParameter\":false,\"Rotation\":\"[0 0 0]\",\"ScalingAsParameter\":false,\"Scaling\":\"[1 1 1]\",\"ObjectsCount\":1},\"PositionAndScaleProperty\":null,\"PositionProperty\":null},\"Children\":[],\"Oid\":10}]}"  evalStr=dsmsi(gcb, 'EvalJson')  sampleTime=-1  globalBlockId=0  objectsBlockId=dsmsi(gcb, 'GetObjectBlockId')  objectsBlockGuiOpen=dsmsi(gcb, 'GetSdoGuiStatus')  dialogIsOpen=0  blockVersion=60  highPrecision=0  validNameBckp=Bounding_Boxes
      settings: SourceProductName=dSPACE MSI Blockset
  Constant : Constant
  Constant1 : Constant  Value=2
  Constant2 : Constant  Value=3
  Constant3 : Constant  Value=4
  Constant4 : Constant  Value=5
  Constant5 : Constant  Value=6
  Constant6 : Constant  Value=7
  Constant7 : Constant  Value=8
  Constant8 : Constant  Value=9
  Constant9 : Constant  Value=10
  EnableBoxVisualization : Subsystem
  Enable_Data_Transfer : Constant
  wires:
  Constant9/1 -> BoundingBox_10/1(Index[])
  Constant8/1 -> BoundingBox_9/1(Index[])
  Constant7/1 -> BoundingBox_8/1(Index[])
  Constant6/1 -> BoundingBox_7/1(Index[])
  Constant5/1 -> BoundingBox_6/1(Index[])
  Constant4/1 -> BoundingBox_5/1(Index[])
  Constant3/1 -> BoundingBox_4/1(Index[])
  Constant2/1 -> BoundingBox_3/1(Index[])
  Constant1/1 -> BoundingBox_2/1(Index[])
  Constant/1 -> BoundingBox_1/1(Index[])
  BoundingBox_1/1(Pos_CoorSysE[m]) -> Bounding_Boxes/2
  BoundingBox_1/2(Angle_CoorSysE[m]) -> Bounding_Boxes/3
  BoundingBox_1/3(Dimensions[m]) -> Bounding_Boxes/4
  Environment_Animation/1 -> EnableBoxVisualization/1(Environment_Animation)
  EnableBoxVisualization/1(BoundigBoxes_Animation) -> BoundingBox_1/2(BoundigBoxes_Animation), BoundingBox_2/2(BoundigBoxes_Animation), BoundingBox_3/2(BoundigBoxes_Animation), BoundingBox_4/2(BoundigBoxes_Animation), BoundingBox_5/2(BoundigBoxes_Animation), BoundingBox_6/2(BoundigBoxes_Animation), BoundingBox_7/2(BoundigBoxes_Animation), BoundingBox_8/2(BoundigBoxes_Animation), BoundingBox_9/2(BoundigBoxes_Animation), BoundingBox_10/2(BoundigBoxes_Animation)
  BoundingBox_2/1(Pos_CoorSysE[m]) -> Bounding_Boxes/5
  BoundingBox_2/2(Angle_CoorSysE[m]) -> Bounding_Boxes/6
  BoundingBox_2/3(Dimensions[m]) -> Bounding_Boxes/7
  BoundingBox_4/3(Dimensions[m]) -> Bounding_Boxes/13
  BoundingBox_4/2(Angle_CoorSysE[m]) -> Bounding_Boxes/12
  BoundingBox_4/1(Pos_CoorSysE[m]) -> Bounding_Boxes/11
  BoundingBox_3/3(Dimensions[m]) -> Bounding_Boxes/10
  BoundingBox_3/2(Angle_CoorSysE[m]) -> Bounding_Boxes/9
  BoundingBox_3/1(Pos_CoorSysE[m]) -> Bounding_Boxes/8
  BoundingBox_7/1(Pos_CoorSysE[m]) -> Bounding_Boxes/20
  BoundingBox_7/2(Angle_CoorSysE[m]) -> Bounding_Boxes/21
  BoundingBox_7/3(Dimensions[m]) -> Bounding_Boxes/22
  BoundingBox_8/1(Pos_CoorSysE[m]) -> Bounding_Boxes/23
  BoundingBox_8/2(Angle_CoorSysE[m]) -> Bounding_Boxes/24
  BoundingBox_8/3(Dimensions[m]) -> Bounding_Boxes/25
  BoundingBox_6/3(Dimensions[m]) -> Bounding_Boxes/19
  BoundingBox_6/2(Angle_CoorSysE[m]) -> Bounding_Boxes/18
  BoundingBox_6/1(Pos_CoorSysE[m]) -> Bounding_Boxes/17
  BoundingBox_5/3(Dimensions[m]) -> Bounding_Boxes/16
  BoundingBox_5/2(Angle_CoorSysE[m]) -> Bounding_Boxes/15
  BoundingBox_5/1(Pos_CoorSysE[m]) -> Bounding_Boxes/14
  BoundingBox_10/3(Dimensions[m]) -> Bounding_Boxes/31
  BoundingBox_10/2(Angle_CoorSysE[m]) -> Bounding_Boxes/30
  BoundingBox_10/1(Pos_CoorSysE[m]) -> Bounding_Boxes/29
  BoundingBox_9/3(Dimensions[m]) -> Bounding_Boxes/28
  BoundingBox_9/2(Angle_CoorSysE[m]) -> Bounding_Boxes/27
  BoundingBox_9/1(Pos_CoorSysE[m]) -> Bounding_Boxes/26
  Enable_Data_Transfer/1 -> Bounding_Boxes/1

== system ASM_AnimationInterface/AnimationInterface/ANIMATION_INTERFACE/Connection_Settings ==
  Environment_Animation : Inport
  Communication_Service : Subsystem  Tag=AnimationInterface_SIL
  Communication_Service_Common_Signals : Subsystem
  Display1 : Display
      settings: Format=decimal (Stored Integer)
  Ethernet_TCP : Subsystem  Tag=AnimationInterface_SIL  Commented=on
  MultiportSwitch{,1..3} (4 alike) : MultiPortSwitch  DataPortOrder=Zero-based contiguous  Inputs=2  zeroidx=on  SaturateOnIntegerOverflow=off  InputSameDT=off
  Sw_CommunicationMethod[0TCP|1ComService] : Constant
  dsmsi_connection_settings_BL1 : dsmsilib/dsmsi_connection_settings_BL1  Priority=10009  rateDividerPort=off  rateDivider=1  application=MotionDesk  reuse=off  source=dsmsilib/dsmsi_connection_settings_BL1  sendObjects=on  comment=Observer  txBufferSize=65507  enableTxBufferSize=off  globalBlockId=dsmsi(gcb, 'GetId')  sourceId=0  numberOfObjectBlocks=dsmsi(gcb, 'CountObjectBlocks')  numberOfGlobalBlocks=dsmsi(gcb, 'CountGlobalBlocks')  numberOfSensorFailureBlocks=dsmsi(gcb, 'CountSensorFailureBlocks')  uuid=7fbc0f5c-1ab5-4f7c-8d42-b98103fe8ad365046cd0-299c-42cd-a0b2-8824978edec42fda6c2b-1778-4453-86b3-4d675bee6ea0  countPipelines=dsmsi(gcb, 'CountPipelines')  debugCom=off  forceInitData=0  blockVersion=60  dialogIsOpen='0'  validNameBckp=dsmsi_connection_settings_BL1  updateFlag=0  Tx_rate_n=1  txRate=1  txRateInputPort=off
      settings: AttributesFormatString=%<comment>  SourceProductName=dSPACE MSI Blockset
  wires:
  Ethernet_TCP/4(Rx_Data) -> MultiportSwitch3/2
  Ethernet_TCP/3(Rx_Length) -> MultiportSwitch2/2
  Ethernet_TCP/2(Tx_Sent_bytes) -> MultiportSwitch1/2
  Ethernet_TCP/1(Connected) -> MultiportSwitch/2
  MultiportSwitch3/1 -> dsmsi_connection_settings_BL1/4
  MultiportSwitch2/1 -> dsmsi_connection_settings_BL1/3
  MultiportSwitch1/1 -> dsmsi_connection_settings_BL1/2
  MultiportSwitch/1 -> dsmsi_connection_settings_BL1/1
  Sw_CommunicationMethod[0TCP|1ComService]/1 -> MultiportSwitch3/1, MultiportSwitch2/1, MultiportSwitch1/1, MultiportSwitch/1
  Communication_Service/4(Rx_Data) -> MultiportSwitch3/3
  Communication_Service/3(Rx_Length) -> MultiportSwitch2/3
  Communication_Service/2(Tx_Sent_bytes) -> MultiportSwitch1/3
  Communication_Service/1(Connected) -> MultiportSwitch/3
  dsmsi_connection_settings_BL1/3 -> Communication_Service/2(Tx_Data), Ethernet_TCP/2(Tx_Data)
  dsmsi_connection_settings_BL1/2 -> Communication_Service/1(Tx_Length), Ethernet_TCP/1(Tx_Length)
  dsmsi_connection_settings_BL1/1 -> Display1/1
  Environment_Animation/1 -> Communication_Service_Common_Signals/1(Environment_Animation)
  Communication_Service_Common_Signals/1(ReferenceTime[s]) -> Communication_Service/3(ReferenceTime[s])
  Communication_Service_Common_Signals/2(Reset[0|1]) -> Communication_Service/4(Reset[0|1])

== system ASM_AnimationInterface/AnimationInterface/ANIMATION_INTERFACE/Data_Streams_Instruments ==
  Environment_Animation : Inport
  Bus Selector2 : BusSelector  OutputSignals=Objects_DataStreams[].DataStream_1[].DataStream_1[],Objects_DataStreams[].DataStream_2[].DataStream_2[],Objects_DataStreams[].DataStream_3[].DataStream_3[],Objects_DataStreams[].DataStream_4[].DataStream_4[],Objects_DataStreams[].DataStream_5[].DataStream_5[],Objects_DataStreams[].DataStream_6[].DataStream_6[],Objects_DataStreams[].DataStream_7[].DataStream_7[],Objects_DataStreams[].DataStream_8[].DataStream_8[]
  Enable_Data_Transfer : Constant
  Objects_DataStreams_Instruments : dsmsilib/dsmsi_simulation_data_objects_BL1  Priority=10001  parameterStr="{\"Version\":1,\"TransformInput\":false,\"EnableInput\":true,\"Objects\":[{\"Name\":\"Obj_DataStream_001\",\"TypeClass\":{\"Name\":\"Signal\",\"Class\":3,\"SignalProperty\":{\"Description\":null,\"Unit\":null,\"Type\":0,\"Length\":1,\"ObjectsCount\":1},\"TransformationProperty\":null,\"PositionAndScaleProperty\":null,\"PositionProperty\":null},\"Children\":[],\"Oid\":1},{\"Name\":\"Obj_DataStream_002\",\"TypeClass\":{\"Name\":\"Signal\",\"Class\":3,\"SignalProperty\":{\"Description\":null,\"Unit\":null,\"Type\":0,\"Length\":1,\"ObjectsCount\":1},\"TransformationProperty\":null,\"PositionAndScaleProperty\":null,\"PositionProperty\":null},\"Children\":[],\"Oid\":2},{\"Name\":\"Obj_DataStream_003\",\"TypeClass\":{\"Name\":\"Signal\",\"Class\":3,\"SignalProperty\":{\"Description\":null,\"Unit\":null,\"Type\":0,\"Length\":1,\"ObjectsCount\":1},\"TransformationProperty\":null,\"PositionAndScaleProperty\":null,\"PositionProperty\":null},\"Children\":[],\"Oid\":3},{\"Name\":\"Obj_DataStream_004\",\"TypeClass\":{\"Name\":\"Signal\",\"Class\":3,\"SignalProperty\":{\"Description\":null,\"Unit\":null,\"Type\":0,\"Length\":1,\"ObjectsCount\":1},\"TransformationProperty\":null,\"PositionAndScaleProperty\":null,\"PositionProperty\":null},\"Children\":[],\"Oid\":4},{\"Name\":\"Obj_DataStream_005\",\"TypeClass\":{\"Name\":\"Signal\",\"Class\":3,\"SignalProperty\":{\"Description\":null,\"Unit\":null,\"Type\":0,\"Length\":1,\"ObjectsCount\":1},\"TransformationProperty\":null,\"PositionAndScaleProperty\":null,\"PositionProperty\":null},\"Children\":[],\"Oid\":5},{\"Name\":\"Obj_DataStream_006\",\"TypeClass\":{\"Name\":\"Signal\",\"Class\":3,\"SignalProperty\":{\"Description\":null,\"Unit\":null,\"Type\":0,\"Length\":1,\"ObjectsCount\":1},\"TransformationProperty\":null,\"PositionAndScaleProperty\":null,\"PositionProperty\":null},\"Children\":[],\"Oid\":6},{\"Name\":\"Obj_DataStream_007\",\"TypeClass\":{\"Name\":\"Signal\",\"Class\":3,\"SignalProperty\":{\"Description\":null,\"Unit\":null,\"Type\":0,\"Length\":1,\"ObjectsCount\":1},\"TransformationProperty\":null,\"PositionAndScaleProperty\":null,\"PositionProperty\":null},\"Children\":[],\"Oid\":7},{\"Name\":\"Obj_DataStream_008\",\"TypeClass\":{\"Name\":\"Signal\",\"Class\":3,\"SignalProperty\":{\"Description\":null,\"Unit\":null,\"Type\":0,\"Length\":1,\"ObjectsCount\":1},\"TransformationProperty\":null,\"PositionAndScaleProperty\":null,\"PositionProperty\":null},\"Children\":[],\"Oid\":8}]}"  evalStr=dsmsi(gcb, 'EvalJson')  sampleTime=-1  globalBlockId=0  objectsBlockId=dsmsi(gcb, 'GetObjectBlockId')  objectsBlockGuiOpen=dsmsi(gcb, 'GetSdoGuiStatus')  dialogIsOpen=0  blockVersion=60  highPrecision=0  validNameBckp=Objects_DataStreams_Instruments
      settings: SourceProductName=dSPACE MSI Blockset
  wires:
  Bus Selector2/5 -> Objects_DataStreams_Instruments/6  "<DataStream_5[]>"
  Bus Selector2/3 -> Objects_DataStreams_Instruments/4  "<DataStream_3[]>"
  Bus Selector2/1 -> Objects_DataStreams_Instruments/2  "<DataStream_1[]>"
  Bus Selector2/8 -> Objects_DataStreams_Instruments/9  "<DataStream_8[]>"
  Bus Selector2/6 -> Objects_DataStreams_Instruments/7  "<DataStream_6[]>"
  Bus Selector2/4 -> Objects_DataStreams_Instruments/5  "<DataStream_4[]>"
  Bus Selector2/7 -> Objects_DataStreams_Instruments/8  "<DataStream_7[]>"
  Bus Selector2/2 -> Objects_DataStreams_Instruments/3  "<DataStream_2[]>"
  Enable_Data_Transfer/1 -> Objects_DataStreams_Instruments/1
  Environment_Animation/1 -> Bus Selector2/1
